simulink model "squawk4_pitchhold"  (R2025a)
settings: Solver=ode45  StartTime=0.0  StopTime=600  MaxStep=0.05  RelTol=1e-6  AbsTol=1e-8
values from neighbouring files (symbols this model uses):
  K_theta = 0    [squawk4_lab.m]
  Keng = diag([1, r2d/u0, r2d, r2d])    [squawk4_lab.m]
  x0 = [10; 0; 0; 0]    [squawk4_lab.m]
undefined symbols (not defined in the file or in its folder): A, B, C, D, u0
settings Model: Creator=rtydf  LastModifiedBy=rtydf

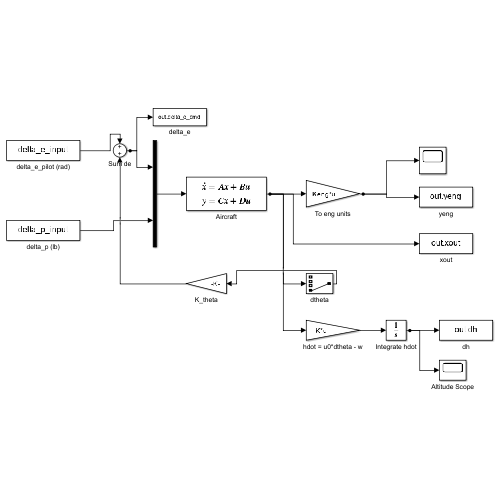
[thumbnail: Simulink's stored preview of the top-level diagram]
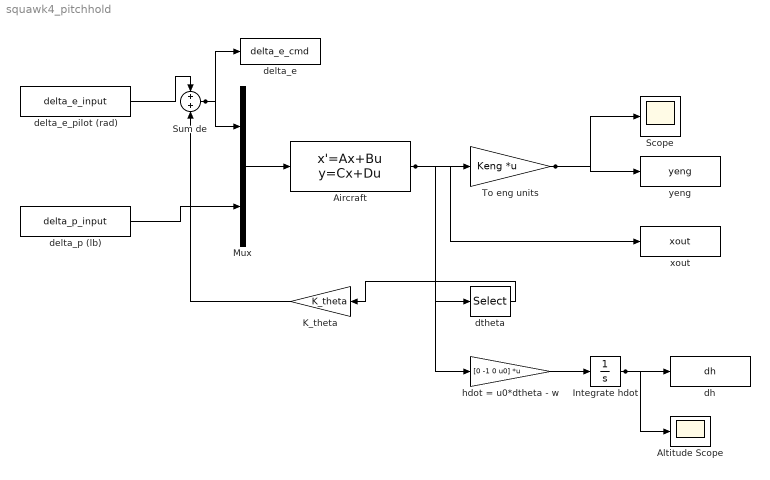
== system squawk4_pitchhold ==
  Aircraft : StateSpace  A=A  B=B  C=C  D=D  InitialCondition=x0
  Altitude Scope : Scope
  Integrate hdot : Integrator
  K_theta : Gain  Gain=K_theta
  Mux : Mux  Inputs=2
  Scope : Scope
  Sum de : Sum
  To eng units : Gain  Gain=Keng  Multiplication=Matrix(K*u)
  delta_e : ToWorkspace  VariableName=delta_e_cmd  SaveFormat=Timeseries  SampleTime=-1
  delta_e_pilot (rad) : FromWorkspace  VariableName=delta_e_input
  delta_p (lb) : FromWorkspace  VariableName=delta_p_input
  dh : ToWorkspace  VariableName=dh  SaveFormat=Timeseries  SampleTime=-1
  dtheta : Selector  InputPortWidth=4  IndexOptions=Index vector (dialog)  Indices=4  OutputSizes=1
  hdot = u0*dtheta - w : Gain  Gain=[0 -1 0 u0]  Multiplication=Matrix(K*u)
  xout : ToWorkspace  VariableName=xout  SaveFormat=Timeseries  SampleTime=-1
  yeng : ToWorkspace  VariableName=yeng  SaveFormat=Timeseries  SampleTime=-1
  wires:
  delta_e_pilot (rad)/1 -> Sum de/1
  Sum de/1 -> Mux/1, delta_e/1
  delta_p (lb)/1 -> Mux/2
  Mux/1 -> Aircraft/1
  Aircraft/1 -> To eng units/1, xout/1, dtheta/1, hdot = u0*dtheta - w/1
  dtheta/1 -> K_theta/1
  K_theta/1 -> Sum de/2
  hdot = u0*dtheta - w/1 -> Integrate hdot/1
  Integrate hdot/1 -> dh/1, Altitude Scope/1
  To eng units/1 -> Scope/1, yeng/1
